simulink library "xps_library"  (Simulink 8.0)
settings: Solver=ode45  SolverMode=SingleTasking  StartTime=0.0  StopTime=10.0  RelTol=1e-3
undefined symbols (not defined in the file): sys_clk, xps_library_software_register_user_data_in
libraries: xbsIndex_r4 x867, simulink x109, dspsigops x81, casper_library_flow_control x68, xps_library x18, casper_library_misc x11
(part 6 of 10)

== system xps_library/ADCs/adc_mkid ==
  conv : Subsystem
      mask help:
      | Converts an (12-bit) unsigned number to 2's complement.
      | This block should eventually be able to handle arbitrary
      | width inputs.
  conv1 : Subsystem
      mask help:
      | Converts an (12-bit) unsigned number to 2's complement.
      | This block should eventually be able to handle arbitrary
      | width inputs.
  conv2 : Subsystem
      mask help:
      | Converts an (12-bit) unsigned number to 2's complement.
      | This block should eventually be able to handle arbitrary
      | width inputs.
  conv3 : Subsystem
      mask help:
      | Converts an (12-bit) unsigned number to 2's complement.
      | This block should eventually be able to handle arbitrary
      | width inputs.
  xps_library_ADCs_adc_mkid_user_data_i0 : xbsIndex_r4/Gateway In  gui_display_data_type=Fixed-point  arith_type=Unsigned  n_bits=12  bin_pt=0  preci_type=Single  exp_width=8  frac_width=24  quantization=Truncate  overflow=Wrap  period=1  dbl_ovrd=off  timing_constraint=None  locs_specified=off  LOCs={}  hdl_port=on  block_type=gatewayin
      settings: infoedit="Gateway in block.  Converts inputs of type Simulink integer, double and fixed point to  Xilinx fixed point type.<P><P>Hardware notes:  In hardware these blocks become top level input ports."  xl_area=[0, 0, 0, 0, 0, 0, 0]  block_version=10.1.3
  xps_library_ADCs_adc_mkid_user_data_i1 : xbsIndex_r4/Gateway In  gui_display_data_type=Fixed-point  arith_type=Unsigned  n_bits=12  bin_pt=0  preci_type=Single  exp_width=8  frac_width=24  quantization=Truncate  overflow=Wrap  period=1  dbl_ovrd=off  timing_constraint=None  locs_specified=off  LOCs={}  hdl_port=on  block_type=gatewayin
      settings: infoedit="Gateway in block.  Converts inputs of type Simulink integer, double and fixed point to  Xilinx fixed point type.<P><P>Hardware notes:  In hardware these blocks become top level input ports."  xl_area=[0, 0, 0, 0, 0, 0, 0]  block_version=10.1.3
  xps_library_ADCs_adc_mkid_user_data_q0 : xbsIndex_r4/Gateway In  gui_display_data_type=Fixed-point  arith_type=Unsigned  n_bits=12  bin_pt=0  preci_type=Single  exp_width=8  frac_width=24  quantization=Truncate  overflow=Wrap  period=1  dbl_ovrd=off  timing_constraint=None  locs_specified=off  LOCs={}  hdl_port=on  block_type=gatewayin
      settings: infoedit="Gateway in block.  Converts inputs of type Simulink integer, double and fixed point to  Xilinx fixed point type.<P><P>Hardware notes:  In hardware these blocks become top level input ports."  xl_area=[0, 0, 0, 0, 0, 0, 0]  block_version=10.1.3
  xps_library_ADCs_adc_mkid_user_data_q1 : xbsIndex_r4/Gateway In  gui_display_data_type=Fixed-point  arith_type=Unsigned  n_bits=12  bin_pt=0  preci_type=Single  exp_width=8  frac_width=24  quantization=Truncate  overflow=Wrap  period=1  dbl_ovrd=off  timing_constraint=None  locs_specified=off  LOCs={}  hdl_port=on  block_type=gatewayin
      settings: infoedit="Gateway in block.  Converts inputs of type Simulink integer, double and fixed point to  Xilinx fixed point type.<P><P>Hardware notes:  In hardware these blocks become top level input ports."  xl_area=[0, 0, 0, 0, 0, 0, 0]  block_version=10.1.3
  xps_library_ADCs_adc_mkid_user_sync : xbsIndex_r4/Gateway In  gui_display_data_type=Fixed-point  arith_type=Boolean  n_bits=1  bin_pt=0  preci_type=Single  exp_width=8  frac_width=24  quantization=Truncate  overflow=Wrap  period=1  dbl_ovrd=off  timing_constraint=None  locs_specified=off  LOCs={}  hdl_port=on  block_type=gatewayin
      settings: infoedit="Gateway in block.  Converts inputs of type Simulink integer, double and fixed point to  Xilinx fixed point type.<P><P>Hardware notes:  In hardware these blocks become top level input ports."  xl_area=[0, 0, 0, 0, 0, 0, 0]  block_version=10.1.3
  data_i0 : Outport
  data_i1 : Outport  Port=2
  data_q0 : Outport  Port=3
  data_q1 : Outport  Port=4
  sync : Outport  Port=5
  wires:
  xps_library_ADCs_adc_mkid_user_sync/1 -> sync/1
  xps_library_ADCs_adc_mkid_user_data_i0/1 -> conv/1(In1)
  conv/1(Out1) -> data_i0/1
  xps_library_ADCs_adc_mkid_user_data_q0/1 -> conv2/1(In1)
  conv2/1(Out1) -> data_q0/1
  xps_library_ADCs_adc_mkid_user_data_i1/1 -> conv1/1(In1)
  conv1/1(Out1) -> data_i1/1
  xps_library_ADCs_adc_mkid_user_data_q1/1 -> conv3/1(In1)
  conv3/1(Out1) -> data_q1/1

== system xps_library/ADCs/adc_mkid_4x ==
  conv : Subsystem
      mask help:
      | Converts an (12-bit) unsigned number to 2's complement.
      | This block should eventually be able to handle arbitrary
      | width inputs.
  conv1 : Subsystem
      mask help:
      | Converts an (12-bit) unsigned number to 2's complement.
      | This block should eventually be able to handle arbitrary
      | width inputs.
  conv2 : Subsystem
      mask help:
      | Converts an (12-bit) unsigned number to 2's complement.
      | This block should eventually be able to handle arbitrary
      | width inputs.
  conv3 : Subsystem
      mask help:
      | Converts an (12-bit) unsigned number to 2's complement.
      | This block should eventually be able to handle arbitrary
      | width inputs.
  conv4 : Subsystem
      mask help:
      | Converts an (12-bit) unsigned number to 2's complement.
      | This block should eventually be able to handle arbitrary
      | width inputs.
  conv5 : Subsystem
      mask help:
      | Converts an (12-bit) unsigned number to 2's complement.
      | This block should eventually be able to handle arbitrary
      | width inputs.
  conv6 : Subsystem
      mask help:
      | Converts an (12-bit) unsigned number to 2's complement.
      | This block should eventually be able to handle arbitrary
      | width inputs.
  conv7 : Subsystem
      mask help:
      | Converts an (12-bit) unsigned number to 2's complement.
      | This block should eventually be able to handle arbitrary
      | width inputs.
  xps_library_ADCs_adc_mkid_4x_user_data_i{0..3} (4 alike) : xbsIndex_r4/Gateway In  gui_display_data_type=Fixed-point  arith_type=Unsigned  n_bits=12  bin_pt=0  preci_type=Single  exp_width=8  frac_width=24  quantization=Truncate  overflow=Wrap  period=1  dbl_ovrd=off  timing_constraint=None  locs_specified=off  LOCs={}  hdl_port=on  block_type=gatewayin
      settings: infoedit="Gateway in block.  Converts inputs of type Simulink integer, double and fixed point to  Xilinx fixed point type.<P><P>Hardware notes:  In hardware these blocks become top level input ports."  xl_area=[0, 0, 0, 0, 0, 0, 0]  block_version=10.1.3
  xps_library_ADCs_adc_mkid_4x_user_data_q{0..3} (4 alike) : xbsIndex_r4/Gateway In  gui_display_data_type=Fixed-point  arith_type=Unsigned  n_bits=12  bin_pt=0  preci_type=Single  exp_width=8  frac_width=24  quantization=Truncate  overflow=Wrap  period=1  dbl_ovrd=off  timing_constraint=None  locs_specified=off  LOCs={}  hdl_port=on  block_type=gatewayin
      settings: infoedit="Gateway in block.  Converts inputs of type Simulink integer, double and fixed point to  Xilinx fixed point type.<P><P>Hardware notes:  In hardware these blocks become top level input ports."  xl_area=[0, 0, 0, 0, 0, 0, 0]  block_version=10.1.3
  xps_library_ADCs_adc_mkid_4x_user_sync : xbsIndex_r4/Gateway In  gui_display_data_type=Fixed-point  arith_type=Boolean  n_bits=1  bin_pt=0  preci_type=Single  exp_width=8  frac_width=24  quantization=Truncate  overflow=Wrap  period=1  dbl_ovrd=off  timing_constraint=None  locs_specified=off  LOCs={}  hdl_port=on  block_type=gatewayin
      settings: infoedit="Gateway in block.  Converts inputs of type Simulink integer, double and fixed point to  Xilinx fixed point type.<P><P>Hardware notes:  In hardware these blocks become top level input ports."  xl_area=[0, 0, 0, 0, 0, 0, 0]  block_version=10.1.3
  data_i0 : Outport
  data_i1 : Outport  Port=2
  data_i2 : Outport  Port=3
  data_i3 : Outport  Port=4
  data_q0 : Outport  Port=5
  data_q1 : Outport  Port=6
  data_q2 : Outport  Port=7
  data_q3 : Outport  Port=8
  sync : Outport  Port=9
  wires:
  xps_library_ADCs_adc_mkid_4x_user_data_q3/1 -> conv7/1(In1)
  conv7/1(Out1) -> data_q3/1
  xps_library_ADCs_adc_mkid_4x_user_data_q2/1 -> conv6/1(In1)
  conv6/1(Out1) -> data_q2/1
  xps_library_ADCs_adc_mkid_4x_user_data_i3/1 -> conv5/1(In1)
  conv5/1(Out1) -> data_i3/1
  xps_library_ADCs_adc_mkid_4x_user_data_i2/1 -> conv4/1(In1)
  conv4/1(Out1) -> data_i2/1
  xps_library_ADCs_adc_mkid_4x_user_sync/1 -> sync/1
  xps_library_ADCs_adc_mkid_4x_user_data_i0/1 -> conv/1(In1)
  conv/1(Out1) -> data_i0/1
  xps_library_ADCs_adc_mkid_4x_user_data_q0/1 -> conv2/1(In1)
  conv2/1(Out1) -> data_q0/1
  xps_library_ADCs_adc_mkid_4x_user_data_i1/1 -> conv1/1(In1)
  conv1/1(Out1) -> data_i1/1
  xps_library_ADCs_adc_mkid_4x_user_data_q1/1 -> conv3/1(In1)
  conv3/1(Out1) -> data_q1/1

== system xps_library/ADCs/adc_sim ==
  sim_adc_data_in : Inport
  adc_bias : Bias  Bias=128  SaturateOnIntegerOverflow=on
  adc_gain : Gain  Gain=128
  overflow_detector : xps_library/ADCs/of_detect_bus  nStreams=8  bit_width=8
  sample0_ds : dspsigops/Downsample  N=8  phase=1  smode=Force single rate  fmode=Maintain input frame rate  ic=0
  sample1_ds : dspsigops/Downsample  N=8  phase=2  smode=Force single rate  fmode=Maintain input frame rate  ic=0
  sample2_ds : dspsigops/Downsample  N=8  phase=3  smode=Force single rate  fmode=Maintain input frame rate  ic=0
  sample3_ds : dspsigops/Downsample  N=8  phase=4  smode=Force single rate  fmode=Maintain input frame rate  ic=0
  sample4_ds : dspsigops/Downsample  N=8  phase=5  smode=Force single rate  fmode=Maintain input frame rate  ic=0
  sample5_ds : dspsigops/Downsample  N=8  phase=6  smode=Force single rate  fmode=Maintain input frame rate  ic=0
  sample6_ds : dspsigops/Downsample  N=8  phase=7  smode=Force single rate  fmode=Maintain input frame rate  ic=0
  sample7_ds : dspsigops/Downsample  N=8  phase=0  smode=Force single rate  fmode=Maintain input frame rate  ic=0
  s0 : Outport
  s1 : Outport  Port=2
  s2 : Outport  Port=3
  s3 : Outport  Port=4
  s4 : Outport  Port=5
  s5 : Outport  Port=6
  s6 : Outport  Port=7
  s7 : Outport  Port=8
  of : Outport  Port=9
  wires:
  sim_adc_data_in/1 -> adc_gain/1
  adc_gain/1 -> adc_bias/1
  overflow_detector/1 -> of/1
  adc_bias/1 -> sample0_ds/1, sample1_ds/1, sample2_ds/1, sample3_ds/1, sample4_ds/1, sample5_ds/1, sample6_ds/1, sample7_ds/1
  sample0_ds/1 -> overflow_detector/1, s0/1
  sample1_ds/1 -> overflow_detector/2, s1/1
  sample2_ds/1 -> overflow_detector/3, s2/1
  sample3_ds/1 -> overflow_detector/4, s3/1
  sample4_ds/1 -> overflow_detector/5, s4/1
  sample5_ds/1 -> overflow_detector/6, s5/1
  sample6_ds/1 -> overflow_detector/7, s6/1
  sample7_ds/1 -> overflow_detector/8, s7/1

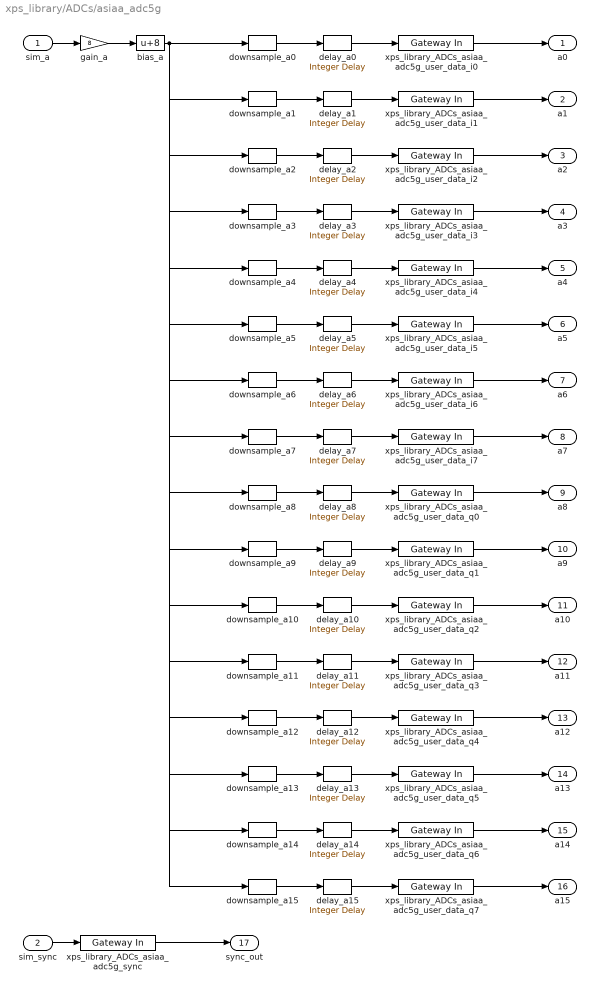
== system xps_library/ADCs/asiaa_adc5g ==
  sim_a : Inport
  sim_sync : Inport  Port=2
  bias_a : Bias  Bias=8  SaturateOnIntegerOverflow=on
  delay_a0 : simulink/Discrete/Integer Delay  NumDelays=2  vinit=0  samptime=-1
  delay_a{1..15} (15 alike) : simulink/Discrete/Integer Delay  NumDelays=1  vinit=0  samptime=-1
  downsample_a0 : dspsigops/Downsample  N=16  phase=0  smode=Allow multirate  fmode=Maintain input frame size  ic=0
  downsample_a1 : dspsigops/Downsample  N=16  phase=1  smode=Allow multirate  fmode=Maintain input frame size  ic=0
  downsample_a10 : dspsigops/Downsample  N=16  phase=10  smode=Allow multirate  fmode=Maintain input frame size  ic=0
  downsample_a11 : dspsigops/Downsample  N=16  phase=11  smode=Allow multirate  fmode=Maintain input frame size  ic=0
  downsample_a12 : dspsigops/Downsample  N=16  phase=12  smode=Allow multirate  fmode=Maintain input frame size  ic=0
  downsample_a13 : dspsigops/Downsample  N=16  phase=13  smode=Allow multirate  fmode=Maintain input frame size  ic=0
  downsample_a14 : dspsigops/Downsample  N=16  phase=14  smode=Allow multirate  fmode=Maintain input frame size  ic=0
  downsample_a15 : dspsigops/Downsample  N=16  phase=15  smode=Allow multirate  fmode=Maintain input frame size  ic=0
  downsample_a2 : dspsigops/Downsample  N=16  phase=2  smode=Allow multirate  fmode=Maintain input frame size  ic=0
  downsample_a3 : dspsigops/Downsample  N=16  phase=3  smode=Allow multirate  fmode=Maintain input frame size  ic=0
  downsample_a4 : dspsigops/Downsample  N=16  phase=4  smode=Allow multirate  fmode=Maintain input frame size  ic=0
  downsample_a5 : dspsigops/Downsample  N=16  phase=5  smode=Allow multirate  fmode=Maintain input frame size  ic=0
  downsample_a6 : dspsigops/Downsample  N=16  phase=6  smode=Allow multirate  fmode=Maintain input frame size  ic=0
  downsample_a7 : dspsigops/Downsample  N=16  phase=7  smode=Allow multirate  fmode=Maintain input frame size  ic=0
  downsample_a8 : dspsigops/Downsample  N=16  phase=8  smode=Allow multirate  fmode=Maintain input frame size  ic=0
  downsample_a9 : dspsigops/Downsample  N=16  phase=9  smode=Allow multirate  fmode=Maintain input frame size  ic=0
  gain_a : Gain  Gain=8  SaturateOnIntegerOverflow=on  OutDataTypeStr=Inherit: Same as input  ParamDataTypeStr=Inherit: Same as input
  xps_library_ADCs_asiaa_adc5g_sync : xbsIndex_r4/Gateway In  gui_display_data_type=Fixed-point  arith_type=Boolean  n_bits=16  bin_pt=14  preci_type=Single  exp_width=8  frac_width=24  quantization="Round  (unbiased: +/- Inf)"  overflow=Saturate  period=1  dbl_ovrd=off  timing_constraint=None  locs_specified=off  LOCs={}  hdl_port=on  block_type=gatewayin
  xps_library_ADCs_asiaa_adc5g_user_data_i{0..7} (8 alike) : xbsIndex_r4/Gateway In  gui_display_data_type=Fixed-point  arith_type=Unsigned  n_bits=4  bin_pt=0  preci_type=Single  exp_width=8  frac_width=24  quantization=Truncate  overflow=Wrap  period=1  dbl_ovrd=off  timing_constraint=None  locs_specified=off  LOCs={}  hdl_port=on  block_type=gatewayin
  xps_library_ADCs_asiaa_adc5g_user_data_q{0..7} (8 alike) : xbsIndex_r4/Gateway In  gui_display_data_type=Fixed-point  arith_type=Unsigned  n_bits=4  bin_pt=0  preci_type=Single  exp_width=8  frac_width=24  quantization=Truncate  overflow=Wrap  period=1  dbl_ovrd=off  timing_constraint=None  locs_specified=off  LOCs={}  hdl_port=on  block_type=gatewayin
  a0 : Outport
  a1 : Outport  Port=2
  a2 : Outport  Port=3
  a3 : Outport  Port=4
  a4 : Outport  Port=5
  a5 : Outport  Port=6
  a6 : Outport  Port=7
  a7 : Outport  Port=8
  a8 : Outport  Port=9
  a9 : Outport  Port=10
  a10 : Outport  Port=11
  a11 : Outport  Port=12
  a12 : Outport  Port=13
  a13 : Outport  Port=14
  a14 : Outport  Port=15
  a15 : Outport  Port=16
  sync_out : Outport  Port=17
  wires:
  sim_a/1 -> gain_a/1
  gain_a/1 -> bias_a/1
  bias_a/1 -> downsample_a0/1, downsample_a1/1, downsample_a2/1, downsample_a3/1, downsample_a4/1, downsample_a5/1, downsample_a6/1, downsample_a7/1, downsample_a8/1, downsample_a9/1, downsample_a10/1, downsample_a11/1, downsample_a12/1, downsample_a13/1, downsample_a14/1, downsample_a15/1
  downsample_a0/1 -> delay_a0/1
  delay_a0/1 -> xps_library_ADCs_asiaa_adc5g_user_data_i0/1
  xps_library_ADCs_asiaa_adc5g_user_data_i0/1 -> a0/1
  downsample_a1/1 -> delay_a1/1
  delay_a1/1 -> xps_library_ADCs_asiaa_adc5g_user_data_i1/1
  xps_library_ADCs_asiaa_adc5g_user_data_i1/1 -> a1/1
  downsample_a2/1 -> delay_a2/1
  delay_a2/1 -> xps_library_ADCs_asiaa_adc5g_user_data_i2/1
  xps_library_ADCs_asiaa_adc5g_user_data_i2/1 -> a2/1
  downsample_a3/1 -> delay_a3/1
  delay_a3/1 -> xps_library_ADCs_asiaa_adc5g_user_data_i3/1
  xps_library_ADCs_asiaa_adc5g_user_data_i3/1 -> a3/1
  downsample_a4/1 -> delay_a4/1
  delay_a4/1 -> xps_library_ADCs_asiaa_adc5g_user_data_i4/1
  xps_library_ADCs_asiaa_adc5g_user_data_i4/1 -> a4/1
  downsample_a5/1 -> delay_a5/1
  delay_a5/1 -> xps_library_ADCs_asiaa_adc5g_user_data_i5/1
  xps_library_ADCs_asiaa_adc5g_user_data_i5/1 -> a5/1
  downsample_a6/1 -> delay_a6/1
  delay_a6/1 -> xps_library_ADCs_asiaa_adc5g_user_data_i6/1
  xps_library_ADCs_asiaa_adc5g_user_data_i6/1 -> a6/1
  downsample_a7/1 -> delay_a7/1
  delay_a7/1 -> xps_library_ADCs_asiaa_adc5g_user_data_i7/1
  xps_library_ADCs_asiaa_adc5g_user_data_i7/1 -> a7/1
  downsample_a8/1 -> delay_a8/1
  delay_a8/1 -> xps_library_ADCs_asiaa_adc5g_user_data_q0/1
  xps_library_ADCs_asiaa_adc5g_user_data_q0/1 -> a8/1
  downsample_a9/1 -> delay_a9/1
  delay_a9/1 -> xps_library_ADCs_asiaa_adc5g_user_data_q1/1
  xps_library_ADCs_asiaa_adc5g_user_data_q1/1 -> a9/1
  downsample_a10/1 -> delay_a10/1
  delay_a10/1 -> xps_library_ADCs_asiaa_adc5g_user_data_q2/1
  xps_library_ADCs_asiaa_adc5g_user_data_q2/1 -> a10/1
  downsample_a11/1 -> delay_a11/1
  delay_a11/1 -> xps_library_ADCs_asiaa_adc5g_user_data_q3/1
  xps_library_ADCs_asiaa_adc5g_user_data_q3/1 -> a11/1
  downsample_a12/1 -> delay_a12/1
  delay_a12/1 -> xps_library_ADCs_asiaa_adc5g_user_data_q4/1
  xps_library_ADCs_asiaa_adc5g_user_data_q4/1 -> a12/1
  downsample_a13/1 -> delay_a13/1
  delay_a13/1 -> xps_library_ADCs_asiaa_adc5g_user_data_q5/1
  xps_library_ADCs_asiaa_adc5g_user_data_q5/1 -> a13/1
  downsample_a14/1 -> delay_a14/1
  delay_a14/1 -> xps_library_ADCs_asiaa_adc5g_user_data_q6/1
  xps_library_ADCs_asiaa_adc5g_user_data_q6/1 -> a14/1
  downsample_a15/1 -> delay_a15/1
  delay_a15/1 -> xps_library_ADCs_asiaa_adc5g_user_data_q7/1
  xps_library_ADCs_asiaa_adc5g_user_data_q7/1 -> a15/1
  sim_sync/1 -> xps_library_ADCs_asiaa_adc5g_sync/1
  xps_library_ADCs_asiaa_adc5g_sync/1 -> sync_out/1

== system xps_library/ADCs/conv ==
  In1 : Inport
  Concat : xbsIndex_r4/Concat  num_inputs=2  dbl_ovrd=off  block_type=concat
      settings: block_version=8.2.02
  Inverter : xbsIndex_r4/Inverter  en=off  latency=0  dbl_ovrd=off  block_type=inv
      settings: xl_area=[0, 0, 0, 0, 0, 0, 0]  block_version=8.2.02
  Reinterpret : xbsIndex_r4/Reinterpret  force_arith_type=on  arith_type="Signed  (2's comp)"  force_bin_pt=on  bin_pt=bit_width-1  block_type=reinterpret
      settings: infoedit="Changes signal type without altering the binary representation.   You can changed the signal between signed and unsigned, and relocate the binary point.<br><br>Hardware notes: In hardware this block costs nothing.<br><br>Example:  Suppose the input is 6 bits wide, signed, with 2 fractional bits, and the output is forced to unsigned with 0 fractional bits.  Then an input of -2.0 (1110.00 in binary 2's complement) becomes an output of 56 (111000 in binary)."  block_version=8.2.02
  Slice : xbsIndex_r4/Slice  nbits=1  boolean_output=off  mode=Upper Bit Location + Width  bit1=0  base1=MSB of Input  bit0=0  base0=LSB of Input  dbl_ovrd=off  block_type=slice
      settings: infoedit="Extracts a given range of bits from each input sample and presents it at the output.  The output type is ordinarily unsigned with binary point at zero, but can be Boolean when the slice is one bit wide.<P><P>Hardware notes: In hardware this block costs nothing."  block_version=8.2.02
  Slice1 : xbsIndex_r4/Slice  nbits=bit_width-1  boolean_output=off  mode=Lower Bit Location + Width  bit1=0  base1=MSB of Input  bit0=0  base0=LSB of Input  dbl_ovrd=off  block_type=slice
      settings: block_version=8.2.02
  Out1 : Outport
  wires:
  Reinterpret/1 -> Out1/1
  Concat/1 -> Reinterpret/1
  Slice1/1 -> Concat/2
  Inverter/1 -> Concat/1
  Slice/1 -> Inverter/1
  In1/1 -> Slice/1, Slice1/1

== system xps_library/ADCs/of1 ==
  s0 : Inport
  s1 : Inport  Port=2
  Compare To Constant1 : simulink/Logic and Bit Operations/Compare To Constant  relop=>  const=2^n_adc_bits-1  LogicOutDataTypeMode=boolean  ZeroCross=off
  Compare To Constant2 : simulink/Logic and Bit Operations/Compare To Constant  relop=>  const=2^n_adc_bits-1  LogicOutDataTypeMode=boolean  ZeroCross=off
  Compare To Constant6 : simulink/Logic and Bit Operations/Compare To Constant  relop=<  const=0  LogicOutDataTypeMode=boolean  ZeroCross=off
  Compare To Constant7 : simulink/Logic and Bit Operations/Compare To Constant  relop=<  const=0  LogicOutDataTypeMode=boolean  ZeroCross=off
  Gain : Gain  Gain=2^(bit_num)
  Logical Operator1 : Logic  Operator=OR  Inputs=4  AllPortsSameDT=off  OutDataTypeStr=boolean
  of : Outport
  wires:
  Gain/1 -> of/1
  s1/1 -> Compare To Constant2/1, Compare To Constant7/1
  Logical Operator1/1 -> Gain/1
  s0/1 -> Compare To Constant1/1, Compare To Constant6/1
  Compare To Constant6/1 -> Logical Operator1/1
  Compare To Constant1/1 -> Logical Operator1/2
  Compare To Constant7/1 -> Logical Operator1/3
  Compare To Constant2/1 -> Logical Operator1/4

== system xps_library/ADCs/of_detect_bus ==
  s0 : Inport
  s1 : Inport  Port=2
  s2 : Inport  Port=3
  s3 : Inport  Port=4
  s4 : Inport  Port=5
  s5 : Inport  Port=6
  s6 : Inport  Port=7
  s7 : Inport  Port=8
  Add : Sum  Inputs=++++
  of0 : xps_library/ADCs/of1  bit_num=0  n_adc_bits=8
  of1 : casper_library_misc/of1  bit_num=0  n_adc_bits=8
  of2 : casper_library_misc/of1  bit_num=0  n_adc_bits=8
  of3 : casper_library_misc/of1  bit_num=0  n_adc_bits=8
  overflow : Outport
  wires:
  s0/1 -> of0/1
  s4/1 -> of0/2
  of0/1 -> Add/1
  s1/1 -> of1/1
  s5/1 -> of1/2
  of1/1 -> Add/2
  s2/1 -> of2/1
  s6/1 -> of2/2
  of2/1 -> Add/3
  s3/1 -> of3/1
  s7/1 -> of3/2
  of3/1 -> Add/4
  Add/1 -> overflow/1

== system xps_library/ADCs/x64_adc ==
  sim0 : Inport
  sim1 : Inport  Port=2
  sim2 : Inport  Port=3
  sim3 : Inport  Port=4
  sim4 : Inport  Port=5
  sim5 : Inport  Port=6
  sim6 : Inport  Port=7
  sim7 : Inport  Port=8
  sim8 : Inport  Port=9
  sim9 : Inport  Port=10
  sim10 : Inport  Port=11
  sim11 : Inport  Port=12
  sim12 : Inport  Port=13
  sim13 : Inport  Port=14
  sim14 : Inport  Port=15
  sim15 : Inport  Port=16
  sim_sync : Inport  Port=17
  adc_rst : Inport  Port=18
  Convert : xbsIndex_r4/Convert  gui_display_data_type=Fixed-point  arith_type=Boolean  n_bits=16  bin_pt=14  float_type=Single  exp_bits=8  fraction_bits=24  quantization=Truncate  overflow=Wrap  en=off  latency=0  dbl_ovrd=off  pipeline=off  block_type=convert
      settings: block_version=11.4
  Terminator : Terminator
  xps_library_ADCs_x64_adc_user_chan_sync : xbsIndex_r4/Gateway In  gui_display_data_type=Fixed-point  arith_type=Unsigned  n_bits=8  bin_pt=0  preci_type=Single  exp_width=8  frac_width=24  quantization="Round  (unbiased: +/- Inf)"  overflow=Saturate  period=1  dbl_ovrd=off  timing_constraint=None  locs_specified=off  LOCs={}  UseAsADC=off  ADCChannel='1'  inherit_from_input=off  hdl_port=on  block_type=gatewayin
      settings: infoedit="Gateway in block.  Converts inputs of type Simulink integer, double and fixed point to  Xilinx fixed point type.<br><br>Hardware notes:  In hardware these blocks become top level input ports."  block_version=11.4
  xps_library_ADCs_x64_adc_user_data{0..15} (16 alike) : xbsIndex_r4/Gateway In  gui_display_data_type=Fixed-point  arith_type="Signed  (2's comp)"  n_bits=12  bin_pt=11  preci_type=Single  exp_width=8  frac_width=24  quantization="Round  (unbiased: +/- Inf)"  overflow=Saturate  period=1  dbl_ovrd=off  timing_constraint=None  locs_specified=off  LOCs={}  UseAsADC=off  ADCChannel='1'  inherit_from_input=off  hdl_port=on  block_type=gatewayin
      settings: infoedit="Gateway in block.  Converts inputs of type Simulink integer, double and fixed point to  Xilinx fixed point type.<br><br>Hardware notes:  In hardware these blocks become top level input ports."  block_version=11.4
  xps_library_ADCs_x64_adc_user_rst : xbsIndex_r4/Gateway Out  inherit_from_input=off  hdl_port=on  timing_constraint=None  locs_specified=off  LOCs={}  UseAsDAC=off  DACChannel='1'  block_type=gatewayout
      settings: infoedit="Gateway out block.  Converts Xilinx fixed point inputs into ouputs of type Simulink integer, double, or fixed point.<br><br>Hardware notes:  In hardware these blocks become top level output ports or are discarded, depending on how they are configured."  block_version=11.4
  dout0 : Outport
  dout1 : Outport  Port=2
  dout2 : Outport  Port=3
  dout3 : Outport  Port=4
  dout4 : Outport  Port=5
  dout5 : Outport  Port=6
  dout6 : Outport  Port=7
  dout7 : Outport  Port=8
  dout8 : Outport  Port=9
  dout9 : Outport  Port=10
  dout10 : Outport  Port=11
  dout11 : Outport  Port=12
  dout12 : Outport  Port=13
  dout13 : Outport  Port=14
  dout14 : Outport  Port=15
  dout15 : Outport  Port=16
  chan_sync : Outport  Port=17
  wires:
  ? -> ?
  ? -> ?
  ? -> ?
  ? -> ?
  sim0/1 -> xps_library_ADCs_x64_adc_user_data0/1
  xps_library_ADCs_x64_adc_user_data0/1 -> dout0/1
  sim2/1 -> xps_library_ADCs_x64_adc_user_data2/1
  xps_library_ADCs_x64_adc_user_data2/1 -> dout2/1
  sim3/1 -> xps_library_ADCs_x64_adc_user_data3/1
  xps_library_ADCs_x64_adc_user_data3/1 -> dout3/1
  sim4/1 -> xps_library_ADCs_x64_adc_user_data4/1
  xps_library_ADCs_x64_adc_user_data4/1 -> dout4/1
  sim5/1 -> xps_library_ADCs_x64_adc_user_data5/1
  xps_library_ADCs_x64_adc_user_data5/1 -> dout5/1
  sim6/1 -> xps_library_ADCs_x64_adc_user_data6/1
  xps_library_ADCs_x64_adc_user_data6/1 -> dout6/1
  sim7/1 -> xps_library_ADCs_x64_adc_user_data7/1
  xps_library_ADCs_x64_adc_user_data7/1 -> dout7/1
  sim8/1 -> xps_library_ADCs_x64_adc_user_data8/1
  xps_library_ADCs_x64_adc_user_data8/1 -> dout8/1
  sim9/1 -> xps_library_ADCs_x64_adc_user_data9/1
  xps_library_ADCs_x64_adc_user_data9/1 -> dout9/1
  sim10/1 -> xps_library_ADCs_x64_adc_user_data10/1
  xps_library_ADCs_x64_adc_user_data10/1 -> dout10/1
  sim11/1 -> xps_library_ADCs_x64_adc_user_data11/1
  xps_library_ADCs_x64_adc_user_data11/1 -> dout11/1
  sim12/1 -> xps_library_ADCs_x64_adc_user_data12/1
  xps_library_ADCs_x64_adc_user_data12/1 -> dout12/1
  sim13/1 -> xps_library_ADCs_x64_adc_user_data13/1
  xps_library_ADCs_x64_adc_user_data13/1 -> dout13/1
  sim14/1 -> xps_library_ADCs_x64_adc_user_data14/1
  xps_library_ADCs_x64_adc_user_data14/1 -> dout14/1
  sim15/1 -> xps_library_ADCs_x64_adc_user_data15/1
  xps_library_ADCs_x64_adc_user_data15/1 -> dout15/1
  sim_sync/1 -> xps_library_ADCs_x64_adc_user_chan_sync/1
  xps_library_ADCs_x64_adc_user_chan_sync/1 -> chan_sync/1
  adc_rst/1 -> Convert/1
  xps_library_ADCs_x64_adc_user_rst/1 -> Terminator/1
  Convert/1 -> xps_library_ADCs_x64_adc_user_rst/1
  sim1/1 -> xps_library_ADCs_x64_adc_user_data1/1
  xps_library_ADCs_x64_adc_user_data1/1 -> dout1/1

== system xps_library/DACs/dac_mkid ==
  data_i0 : Inport
  data_i1 : Inport  Port=2
  data_q0 : Inport  Port=3
  data_q1 : Inport  Port=4
  sync_i : Inport  Port=5
  sync_q : Inport  Port=6
  sdenb : Inport  Port=7
  config10Data : Inport  Port=8
  reset : Inport  Port=9
  Convert{,1..3} (4 alike) : xbsIndex_r4/Convert  gui_display_data_type=Fixed-point  arith_type="Signed  (2's comp)"  n_bits=16  bin_pt=15  float_type=Single  exp_bits=8  fraction_bits=24  quantization=Truncate  overflow=Wrap  en=off  latency=0  dbl_ovrd=off  pipeline=off  block_type=convert
      settings: block_version=10.1.3
  Inverter : xbsIndex_r4/Inverter  en=off  latency=0  dbl_ovrd=off  block_type=inv
  Subsystem : Subsystem
  convert_not_reset : xbsIndex_r4/Convert  gui_display_data_type=Fixed-point  arith_type=Boolean  n_bits=16  bin_pt=0  float_type=Single  exp_bits=8  fraction_bits=24  quantization=Truncate  overflow=Wrap  en=off  latency=0  dbl_ovrd=off  pipeline=off  block_type=convert
      settings: block_version=10.1.3
  convert_not_sdenb_i : xbsIndex_r4/Convert  gui_display_data_type=Fixed-point  arith_type=Boolean  n_bits=16  bin_pt=0  float_type=Single  exp_bits=8  fraction_bits=24  quantization=Truncate  overflow=Wrap  en=off  latency=0  dbl_ovrd=off  pipeline=off  block_type=convert
      settings: block_version=10.1.3
  convert_not_sdenb_q : xbsIndex_r4/Convert  gui_display_data_type=Fixed-point  arith_type=Boolean  n_bits=16  bin_pt=0  float_type=Single  exp_bits=8  fraction_bits=24  quantization=Truncate  overflow=Wrap  en=off  latency=0  dbl_ovrd=off  pipeline=off  block_type=convert
      settings: block_version=10.1.3
  convert_sclk : xbsIndex_r4/Convert  gui_display_data_type=Fixed-point  arith_type=Boolean  n_bits=16  bin_pt=0  float_type=Single  exp_bits=8  fraction_bits=24  quantization=Truncate  overflow=Wrap  en=off  latency=0  dbl_ovrd=off  pipeline=off  block_type=convert
      settings: block_version=10.1.3
  convert_sdi : xbsIndex_r4/Convert  gui_display_data_type=Fixed-point  arith_type=Boolean  n_bits=16  bin_pt=0  float_type=Single  exp_bits=8  fraction_bits=24  quantization=Truncate  overflow=Wrap  en=off  latency=0  dbl_ovrd=off  pipeline=off  block_type=convert
      settings: block_version=10.1.3
  convert_sync_i : xbsIndex_r4/Convert  gui_display_data_type=Fixed-point  arith_type=Boolean  n_bits=16  bin_pt=0  float_type=Single  exp_bits=8  fraction_bits=24  quantization=Truncate  overflow=Wrap  en=off  latency=0  dbl_ovrd=off  pipeline=off  block_type=convert
      settings: block_version=10.1.3
  convert_sync_q : xbsIndex_r4/Convert  gui_display_data_type=Fixed-point  arith_type=Boolean  n_bits=16  bin_pt=0  float_type=Single  exp_bits=8  fraction_bits=24  quantization=Truncate  overflow=Wrap  en=off  latency=0  dbl_ovrd=off  pipeline=off  block_type=convert
      settings: block_version=10.1.3
  xps_library_DACs_dac_mkid_dac_data_i0 : xbsIndex_r4/Gateway Out  hdl_port=on  timing_constraint=None  locs_specified=off  LOCs={}  block_type=gatewayout  OutDataTypeMode=boolean
      settings: infoedit="Gateway out block.  Converts Xilinx fixed point inputs into ouputs of type Simulink integer, double, or fixed point.<P><P>Hardware notes:  In hardware these blocks become top level output ports or are discarded, depending on how they are configured."  block_version=10.1.3
  xps_library_DACs_dac_mkid_dac_data_i1 : xbsIndex_r4/Gateway Out  hdl_port=on  timing_constraint=None  locs_specified=off  LOCs={}  block_type=gatewayout
      settings: infoedit="Gateway out block.  Converts Xilinx fixed point inputs into ouputs of type Simulink integer, double, or fixed point.<P><P>Hardware notes:  In hardware these blocks become top level output ports or are discarded, depending on how they are configured."  block_version=10.1.3
  xps_library_DACs_dac_mkid_dac_data_q0 : xbsIndex_r4/Gateway Out  hdl_port=on  timing_constraint=None  locs_specified=off  LOCs={}  block_type=gatewayout
      settings: infoedit="Gateway out block.  Converts Xilinx fixed point inputs into ouputs of type Simulink integer, double, or fixed point.<P><P>Hardware notes:  In hardware these blocks become top level output ports or are discarded, depending on how they are configured."  block_version=10.1.3
  xps_library_DACs_dac_mkid_dac_data_q1 : xbsIndex_r4/Gateway Out  hdl_port=on  timing_constraint=None  locs_specified=off  LOCs={}  block_type=gatewayout
      settings: infoedit="Gateway out block.  Converts Xilinx fixed point inputs into ouputs of type Simulink integer, double, or fixed point.<P><P>Hardware notes:  In hardware these blocks become top level output ports or are discarded, depending on how they are configured."  block_version=10.1.3
  xps_library_DACs_dac_mkid_dac_sync_i : xbsIndex_r4/Gateway Out  hdl_port=on  timing_constraint=None  locs_specified=off  LOCs={}  block_type=gatewayout
      settings: infoedit="Gateway out block.  Converts Xilinx fixed point inputs into ouputs of type Simulink integer, double, or fixed point.<P><P>Hardware notes:  In hardware these blocks become top level output ports or are discarded, depending on how they are configured."  block_version=10.1.3
  xps_library_DACs_dac_mkid_dac_sync_q : xbsIndex_r4/Gateway Out  hdl_port=on  timing_constraint=None  locs_specified=off  LOCs={}  block_type=gatewayout
      settings: infoedit="Gateway out block.  Converts Xilinx fixed point inputs into ouputs of type Simulink integer, double, or fixed point.<P><P>Hardware notes:  In hardware these blocks become top level output ports or are discarded, depending on how they are configured."  block_version=10.1.3
  xps_library_DACs_dac_mkid_not_reset : xbsIndex_r4/Gateway Out  hdl_port=on  timing_constraint=None  locs_specified=off  LOCs={}  block_type=gatewayout
      settings: infoedit="Gateway out block.  Converts Xilinx fixed point inputs into ouputs of type Simulink integer, double, or fixed point.<P><P>Hardware notes:  In hardware these blocks become top level output ports or are discarded, depending on how they are configured."  block_version=10.1.3
  xps_library_DACs_dac_mkid_not_sdenb_i : xbsIndex_r4/Gateway Out  hdl_port=on  timing_constraint=None  locs_specified=off  LOCs={}  block_type=gatewayout
      settings: infoedit="Gateway out block.  Converts Xilinx fixed point inputs into ouputs of type Simulink integer, double, or fixed point.<P><P>Hardware notes:  In hardware these blocks become top level output ports or are discarded, depending on how they are configured."  block_version=10.1.3
  xps_library_DACs_dac_mkid_not_sdenb_q : xbsIndex_r4/Gateway Out  hdl_port=on  timing_constraint=None  locs_specified=off  LOCs={}  block_type=gatewayout
      settings: infoedit="Gateway out block.  Converts Xilinx fixed point inputs into ouputs of type Simulink integer, double, or fixed point.<P><P>Hardware notes:  In hardware these blocks become top level output ports or are discarded, depending on how they are configured."  block_version=10.1.3
  xps_library_DACs_dac_mkid_sclk : xbsIndex_r4/Gateway Out  hdl_port=on  timing_constraint=None  locs_specified=off  LOCs={}  block_type=gatewayout
      settings: infoedit="Gateway out block.  Converts Xilinx fixed point inputs into ouputs of type Simulink integer, double, or fixed point.<P><P>Hardware notes:  In hardware these blocks become top level output ports or are discarded, depending on how they are configured."  block_version=10.1.3
  xps_library_DACs_dac_mkid_sdi : xbsIndex_r4/Gateway Out  hdl_port=on  timing_constraint=None  locs_specified=off  LOCs={}  block_type=gatewayout
      settings: infoedit="Gateway out block.  Converts Xilinx fixed point inputs into ouputs of type Simulink integer, double, or fixed point.<P><P>Hardware notes:  In hardware these blocks become top level output ports or are discarded, depending on how they are configured."  block_version=10.1.3
  wires:
  sync_i/1 -> convert_sync_i/1
  convert_sync_i/1 -> xps_library_DACs_dac_mkid_dac_sync_i/1
  sync_q/1 -> convert_sync_q/1
  convert_sync_q/1 -> xps_library_DACs_dac_mkid_dac_sync_q/1
  data_i0/1 -> Convert/1
  Convert/1 -> xps_library_DACs_dac_mkid_dac_data_i0/1
  data_i1/1 -> Convert1/1
  Convert1/1 -> xps_library_DACs_dac_mkid_dac_data_i1/1
  data_q0/1 -> Convert2/1
  Convert2/1 -> xps_library_DACs_dac_mkid_dac_data_q0/1
  data_q1/1 -> Convert3/1
  Convert3/1 -> xps_library_DACs_dac_mkid_dac_data_q1/1
  convert_not_sdenb_i/1 -> xps_library_DACs_dac_mkid_not_sdenb_i/1
  convert_not_sdenb_q/1 -> xps_library_DACs_dac_mkid_not_sdenb_q/1
  convert_sdi/1 -> xps_library_DACs_dac_mkid_sdi/1
  convert_sclk/1 -> xps_library_DACs_dac_mkid_sclk/1
  config10Data/1 -> Subsystem/1(pDataIn)
  Subsystem/1(sDataOut) -> convert_sdi/1
  Subsystem/3(sclk) -> convert_sclk/1
  Subsystem/2(enableOut) -> convert_not_sdenb_i/1, convert_not_sdenb_q/1
  sdenb/1 -> Subsystem/2(start)
  reset/1 -> Inverter/1
  Inverter/1 -> convert_not_reset/1
  convert_not_reset/1 -> xps_library_DACs_dac_mkid_not_reset/1

== system xps_library/DACs/dac_mkid_4x ==
  data_i0 : Inport
  data_i1 : Inport  Port=2
  data_i2 : Inport  Port=3
  data_i3 : Inport  Port=4
  data_q0 : Inport  Port=5
  data_q1 : Inport  Port=6
  data_q2 : Inport  Port=7
  data_q3 : Inport  Port=8
  sync_i : Inport  Port=9
  sync_q : Inport  Port=10
  sdenb : Inport  Port=11
  config10Data : Inport  Port=12
  reset : Inport  Port=13
  Convert{,1..7} (8 alike) : xbsIndex_r4/Convert  gui_display_data_type=Fixed-point  arith_type="Signed  (2's comp)"  n_bits=16  bin_pt=15  float_type=Single  exp_bits=8  fraction_bits=24  quantization=Truncate  overflow=Wrap  en=off  latency=0  dbl_ovrd=off  pipeline=off  block_type=convert
      settings: block_version=10.1.3
  Inverter : xbsIndex_r4/Inverter  en=off  latency=0  dbl_ovrd=off  block_type=inv
  Subsystem : Subsystem
  convert_not_reset : xbsIndex_r4/Convert  gui_display_data_type=Fixed-point  arith_type=Boolean  n_bits=16  bin_pt=0  float_type=Single  exp_bits=8  fraction_bits=24  quantization=Truncate  overflow=Wrap  en=off  latency=0  dbl_ovrd=off  pipeline=off  block_type=convert
      settings: block_version=10.1.3
  convert_not_sdenb_i : xbsIndex_r4/Convert  gui_display_data_type=Fixed-point  arith_type=Boolean  n_bits=16  bin_pt=0  float_type=Single  exp_bits=8  fraction_bits=24  quantization=Truncate  overflow=Wrap  en=off  latency=0  dbl_ovrd=off  pipeline=off  block_type=convert
      settings: block_version=10.1.3
  convert_not_sdenb_q : xbsIndex_r4/Convert  gui_display_data_type=Fixed-point  arith_type=Boolean  n_bits=16  bin_pt=0  float_type=Single  exp_bits=8  fraction_bits=24  quantization=Truncate  overflow=Wrap  en=off  latency=0  dbl_ovrd=off  pipeline=off  block_type=convert
      settings: block_version=10.1.3
  convert_sclk : xbsIndex_r4/Convert  gui_display_data_type=Fixed-point  arith_type=Boolean  n_bits=16  bin_pt=0  float_type=Single  exp_bits=8  fraction_bits=24  quantization=Truncate  overflow=Wrap  en=off  latency=0  dbl_ovrd=off  pipeline=off  block_type=convert
      settings: block_version=10.1.3
  convert_sdi : xbsIndex_r4/Convert  gui_display_data_type=Fixed-point  arith_type=Boolean  n_bits=16  bin_pt=0  float_type=Single  exp_bits=8  fraction_bits=24  quantization=Truncate  overflow=Wrap  en=off  latency=0  dbl_ovrd=off  pipeline=off  block_type=convert
      settings: block_version=10.1.3
  convert_sync_i : xbsIndex_r4/Convert  gui_display_data_type=Fixed-point  arith_type=Boolean  n_bits=16  bin_pt=0  float_type=Single  exp_bits=8  fraction_bits=24  quantization=Truncate  overflow=Wrap  en=off  latency=0  dbl_ovrd=off  pipeline=off  block_type=convert
      settings: block_version=10.1.3
  convert_sync_q : xbsIndex_r4/Convert  gui_display_data_type=Fixed-point  arith_type=Boolean  n_bits=16  bin_pt=0  float_type=Single  exp_bits=8  fraction_bits=24  quantization=Truncate  overflow=Wrap  en=off  latency=0  dbl_ovrd=off  pipeline=off  block_type=convert
      settings: block_version=10.1.3
  xps_library_DACs_dac_mkid_4x_not_reset : xbsIndex_r4/Gateway Out  hdl_port=on  timing_constraint=None  locs_specified=off  LOCs={}  block_type=gatewayout
      settings: infoedit="Gateway out block.  Converts Xilinx fixed point inputs into ouputs of type Simulink integer, double, or fixed point.<P><P>Hardware notes:  In hardware these blocks become top level output ports or are discarded, depending on how they are configured."  block_version=10.1.3
  xps_library_DACs_dac_mkid_4x_not_sdenb_i : xbsIndex_r4/Gateway Out  hdl_port=on  timing_constraint=None  locs_specified=off  LOCs={}  block_type=gatewayout
      settings: infoedit="Gateway out block.  Converts Xilinx fixed point inputs into ouputs of type Simulink integer, double, or fixed point.<P><P>Hardware notes:  In hardware these blocks become top level output ports or are discarded, depending on how they are configured."  block_version=10.1.3
  xps_library_DACs_dac_mkid_4x_not_sdenb_q : xbsIndex_r4/Gateway Out  hdl_port=on  timing_constraint=None  locs_specified=off  LOCs={}  block_type=gatewayout
      settings: infoedit="Gateway out block.  Converts Xilinx fixed point inputs into ouputs of type Simulink integer, double, or fixed point.<P><P>Hardware notes:  In hardware these blocks become top level output ports or are discarded, depending on how they are configured."  block_version=10.1.3
  xps_library_DACs_dac_mkid_4x_sclk : xbsIndex_r4/Gateway Out  hdl_port=on  timing_constraint=None  locs_specified=off  LOCs={}  block_type=gatewayout
      settings: infoedit="Gateway out block.  Converts Xilinx fixed point inputs into ouputs of type Simulink integer, double, or fixed point.<P><P>Hardware notes:  In hardware these blocks become top level output ports or are discarded, depending on how they are configured."  block_version=10.1.3
  xps_library_DACs_dac_mkid_4x_sdi : xbsIndex_r4/Gateway Out  hdl_port=on  timing_constraint=None  locs_specified=off  LOCs={}  block_type=gatewayout
      settings: infoedit="Gateway out block.  Converts Xilinx fixed point inputs into ouputs of type Simulink integer, double, or fixed point.<P><P>Hardware notes:  In hardware these blocks become top level output ports or are discarded, depending on how they are configured."  block_version=10.1.3
  xps_library_DACs_dac_mkid_4x_user_data_i{0..3} (4 alike) : xbsIndex_r4/Gateway Out  hdl_port=on  timing_constraint=None  locs_specified=off  LOCs={}  block_type=gatewayout
      settings: infoedit="Gateway out block.  Converts Xilinx fixed point inputs into ouputs of type Simulink integer, double, or fixed point.<P><P>Hardware notes:  In hardware these blocks become top level output ports or are discarded, depending on how they are configured."  block_version=10.1.3
  xps_library_DACs_dac_mkid_4x_user_data_q{0..3} (4 alike) : xbsIndex_r4/Gateway Out  hdl_port=on  timing_constraint=None  locs_specified=off  LOCs={}  block_type=gatewayout
      settings: infoedit="Gateway out block.  Converts Xilinx fixed point inputs into ouputs of type Simulink integer, double, or fixed point.<P><P>Hardware notes:  In hardware these blocks become top level output ports or are discarded, depending on how they are configured."  block_version=10.1.3
  xps_library_DACs_dac_mkid_4x_user_sync_i : xbsIndex_r4/Gateway Out  hdl_port=on  timing_constraint=None  locs_specified=off  LOCs={}  block_type=gatewayout
      settings: infoedit="Gateway out block.  Converts Xilinx fixed point inputs into ouputs of type Simulink integer, double, or fixed point.<P><P>Hardware notes:  In hardware these blocks become top level output ports or are discarded, depending on how they are configured."  block_version=10.1.3
  xps_library_DACs_dac_mkid_4x_user_sync_q : xbsIndex_r4/Gateway Out  hdl_port=on  timing_constraint=None  locs_specified=off  LOCs={}  block_type=gatewayout
      settings: infoedit="Gateway out block.  Converts Xilinx fixed point inputs into ouputs of type Simulink integer, double, or fixed point.<P><P>Hardware notes:  In hardware these blocks become top level output ports or are discarded, depending on how they are configured."  block_version=10.1.3
  wires:
  convert_not_sdenb_i/1 -> xps_library_DACs_dac_mkid_4x_not_sdenb_i/1
  convert_not_sdenb_q/1 -> xps_library_DACs_dac_mkid_4x_not_sdenb_q/1
  convert_sdi/1 -> xps_library_DACs_dac_mkid_4x_sdi/1
  convert_sclk/1 -> xps_library_DACs_dac_mkid_4x_sclk/1
  config10Data/1 -> Subsystem/1(pDataIn)
  Subsystem/1(sDataOut) -> convert_sdi/1
  Subsystem/3(sclk) -> convert_sclk/1
  Subsystem/2(enableOut) -> convert_not_sdenb_i/1, convert_not_sdenb_q/1
  sdenb/1 -> Subsystem/2(start)
  reset/1 -> Inverter/1
  Inverter/1 -> convert_not_reset/1
  convert_not_reset/1 -> xps_library_DACs_dac_mkid_4x_not_reset/1
  data_i0/1 -> Convert/1
  Convert/1 -> xps_library_DACs_dac_mkid_4x_user_data_i0/1
  data_i1/1 -> Convert1/1
  data_i2/1 -> Convert2/1
  Convert2/1 -> xps_library_DACs_dac_mkid_4x_user_data_i2/1
  Convert1/1 -> xps_library_DACs_dac_mkid_4x_user_data_i1/1
  data_i3/1 -> Convert3/1
  Convert3/1 -> xps_library_DACs_dac_mkid_4x_user_data_i3/1
  data_q0/1 -> Convert4/1
  Convert4/1 -> xps_library_DACs_dac_mkid_4x_user_data_q0/1
  data_q1/1 -> Convert5/1
  Convert5/1 -> xps_library_DACs_dac_mkid_4x_user_data_q1/1
  data_q2/1 -> Convert6/1
  Convert6/1 -> xps_library_DACs_dac_mkid_4x_user_data_q2/1
  data_q3/1 -> Convert7/1
  Convert7/1 -> xps_library_DACs_dac_mkid_4x_user_data_q3/1
  sync_i/1 -> convert_sync_i/1
  convert_sync_i/1 -> xps_library_DACs_dac_mkid_4x_user_sync_i/1
  sync_q/1 -> convert_sync_q/1
  convert_sync_q/1 -> xps_library_DACs_dac_mkid_4x_user_sync_q/1

== system xps_library/Shared BRAM/calc_add ==
  note: If reading/writing words
      | smaller than 32 bits,
      | change address so
      | that addressing is
      | big endian instead of
      | little, otherwise
      | pass through
  note: Use behavioural HDL
      | so that gets optimised
      | to minimum logic
  in : Inport
  add_sub : xbsIndex_r4/AddSub  mode=Subtraction  use_carryin=off  use_carryout=off  en=off  latency=0  precision=User Defined  arith_type=Unsigned  n_bits=max(1, log2(32/data_width))  bin_pt=0  quantization=Truncate  overflow=Wrap  dbl_ovrd=off  use_behavioral_HDL=on  hw_selection=Fabric  pipelined=off  block_type=addsub
  concat : xbsIndex_r4/Concat  num_inputs=2  dbl_ovrd=off  block_type=concat
  const : xbsIndex_r4/Constant  const=max(0, 32/data_width-1)  gui_display_data_type=Fixed-point  arith_type=Unsigned  n_bits=max(1, log2(32/data_width))  bin_pt=0  preci_type=Single  exp_width=8  frac_width=24  explicit_period=on  period=sample_rate  equ=P=C  opselect=C  inp2=PCIN>>17  opr=+  inp1=P  carry=CIN  dbl_ovrd=off  block_type=constant
      settings: block_version=11.4
  convert_addr : xbsIndex_r4/Convert  gui_display_data_type=Fixed-point  arith_type=Unsigned  n_bits=addr_width  bin_pt=0  float_type=Single  exp_bits=8  fraction_bits=24  quantization=Truncate  overflow=Wrap  en=off  latency=0  dbl_ovrd=off  pipeline=off  block_type=convert
      settings: xl_area=[0, 0, 0, 0, 0, 0, 0]
  lsw : xbsIndex_r4/Slice  nbits=max(1, log2(32/data_width))  boolean_output=off  mode=Lower Bit Location + Width  bit1=0  base1=MSB of Input  bit0=0  base0=LSB of Input  dbl_ovrd=off  block_type=slice
  manipulate : xbsIndex_r4/Constant  const=min(1, floor(32/data_width) - 1)  gui_display_data_type=Fixed-point  arith_type=Unsigned  n_bits=1  bin_pt=0  preci_type=Single  exp_width=8  frac_width=24  explicit_period=on  period=sample_rate  equ=P=C  opselect=C  inp2=PCIN>>17  opr=+  inp1=P  carry=CIN  dbl_ovrd=off  block_type=constant
      settings: block_version=11.4
  msw : xbsIndex_r4/Slice  nbits=addr_width - max(1, log2(32/data_width))  boolean_output=off  mode=Upper Bit Location + Width  bit1=0  base1=MSB of Input  bit0=0  base0=LSB of Input  dbl_ovrd=off  block_type=slice
  mux : xbsIndex_r4/Mux  inputs=2  en=off  latency=0  precision=Full  arith_type=Unsigned  n_bits=16  bin_pt=14  quantization=Truncate  overflow=Wrap  dbl_ovrd=off  block_type=mux
      settings: block_version=11.4
  out : Outport
  wires:
  in/1 -> convert_addr/1
  add_sub/1 -> concat/2
  msw/1 -> concat/1
  concat/1 -> mux/3
  manipulate/1 -> mux/1
  mux/1 -> out/1
  lsw/1 -> add_sub/2
  const/1 -> add_sub/1
  convert_addr/1 -> lsw/1, msw/1, mux/2
